simulink model "microduck_nonlinear_state_feedback"  (R2026b)
settings: Solver=ode15s  StopTime=r.test.duration  MaxStep=r.p.cfg.sim.maxStep  RelTol=r.p.cfg.sim.relTol  AbsTol=r.p.cfg.sim.absTol
PreLoadFcn:
  | root=fileparts(get_param(bdroot,'FileName')); addpath(root,fullfile(root,'helpers')); md_expanded_cache;
PostLoadFcn:
  | md_sf_apply(bdroot);
InitFcn:
  | md_sf_apply(bdroot);
model workspace (MAT data in the model file):
  G11 = [-0.6  0; 0  -0.6]
  G12 = -12
  G13 = -4000
  G14 = [-0.6  0; 0  -0.6]
  G15 = -12
  G16 = -4000
  G17 = [-0.6  0; 0  -0.6]
  G18 = -12
  G19 = -4000
  G20 = [-0.6  0; 0  -0.6]
  G21 = -12
  G22 = -4000
  G23 = [-0.6  0; 0  -0.6]
  G24 = -12
  G25 = -4000
  G26 = [-0.6  0; 0  -0.6]
  G27 = -12
  G28 = -4000
  G29 = [-0.6  0; 0  -0.6]
  G30 = -12
  G31 = -4000
  G32 = [-0.6  0; 0  -0.6]
  G33 = -12
  G34 = -4000
  G35 = [0  0  0  0  0  0  0  0; 0  0  0  0  0  0  0  0; 0  0  0  0  0  0  0  0; 0  0  0  0  0  0  0  0; 0  0  0  0  0  0  0  0; 0  0  0  0  0  0  0  0; 1  0  0  0  0  0  0  0; 0  1  0  0  0  0  0  0; 0  0  1  0  0  0  0  0; 0  0  0  1  0  0  0  0; 0  0  0  0  1  0  0  0; 0  0  0  0  0  1  0  0; 0  0  0  0  0  0  1  0; 0  0  0  0  0  0  0  1]
  G36 = [0  0  0  0  0  0  0  0; 0  0  0  0  0  0  0  0; 0  0  0  0  0  0  0  0; 0  0  0  0  0  0  0  0; 0  0  0  0  0  0  0  0; 0  0  0  0  0  0  0  0; 0.053  0  0  0  0  0  0  0; 0  0.053  0  0  0  0  0  0; 0  0  0.053  0  0  0  0  0; 0  0  0  0.053  0  0  0  0; 0  0  0  0  0.053  0  0  0; 0  0  0  0  0  0.053  0  0; 0  0  0  0  0  0  0.053  0; 0  0  0  0  0  0  0  0.053]
  G39 = [33.3333333333  0  0  0  0  0  0  0; 0  33.3333333333  0  0  0  0  0  0; 0  0  33.3333333333  0  0  0  0  0; 0  0  0  33.3333333333  0  0  0  0; 0  0  0  0  33.3333333333  0  0  0; 0  0  0  0  0  33.3333333333  0  0; 0  0  0  0  0  0  33.3333333333  0; 0  0  0  0  0  0  0  33.3333333333]
  G40 = [0  0  0  0  0  0  1  0  0  0  0  0  0  0; 0  0  0  0  0  0  0  1  0  0  0  0  0  0; 0  0  0  0  0  0  0  0  1  0  0  0  0  0; 0  0  0  0  0  0  0  0  0  1  0  0  0  0; 0  0  0  0  0  0  0  0  0  0  1  0  0  0; 0  0  0  0  0  0  0  0  0  0  0  1  0  0; 0  0  0  0  0  0  0  0  0  0  0  0  1  0; 0  0  0  0  0  0  0  0  0  0  0  0  0  1]
  G41 = [0  0  0  0  0  0  1  0  0  0  0  0  0  0; 0  0  0  0  0  0  0  1  0  0  0  0  0  0; 0  0  0  0  0  0  0  0  1  0  0  0  0  0; 0  0  0  0  0  0  0  0  0  1  0  0  0  0; 0  0  0  0  0  0  0  0  0  0  1  0  0  0; 0  0  0  0  0  0  0  0  0  0  0  1  0  0; 0  0  0  0  0  0  0  0  0  0  0  0  1  0; 0  0  0  0  0  0  0  0  0  0  0  0  0  1]
  Kd_servo = [0  0  0  0  0  0  0  0; 0  0  0  0  0  0  0  0; 0  0  0  0  0  0  0  0; 0  0  0  0  0  0  0  0; 0  0  0  0  0  0  0  0; 0  0  0  0  0  0  0  0; 0  0  0  0  0  0  0  0; 0  0  0  0  0  0  0  0]
  Kp_servo = [0.55  0  0  0  0  0  0  0; 0  0.55  0  0  0  0  0  0; 0  0  0.55  0  0  0  0  0; 0  0  0  0.55  0  0  0  0; 0  0  0  0  0.55  0  0  0; 0  0  0  0  0  0.55  0  0; 0  0  0  0  0  0  0.55  0; 0  0  0  0  0  0  0  0.55]
  c10 = 0
  c11 = 0
  c13 = 0
  c14 = 0
  c16 = 0
  c17 = 0
  c19 = 0
  c20 = 0
  c22 = 0
  c23 = 0
  c25 = 0
  c26 = 0
  c4 = 0
  c5 = 0
  c7 = 0
  c8 = 0
  g_world = [0; 0; -9.81]
  push_wrench = [1; 0; 0; 0; 0; 0]
  r.p.cfg.robot.gravity = [0; 0; -9.81]
  r.p.cfg.robot.hipHalfSpacing = 0.04
  r.p.cfg.robot.hipPitchDrop = 0.01
  r.p.cfg.robot.thighLength = 0.05
  r.p.cfg.robot.shinLength = 0.05
  r.p.cfg.robot.thighWidth = 0.025
  r.p.cfg.robot.shinWidth = 0.022
  r.p.cfg.robot.footLength = 0.054
  r.p.cfg.robot.footWidth = 0.041
  r.p.cfg.robot.footThickness = 0.012
  r.p.cfg.robot.soleDepth = 0.018
  r.p.cfg.robot.torsoDimensions = [0.09; 0.1; 0.14]
  r.p.cfg.robot.imuOffset = [0; 0; 0.05]
  r.p.cfg.robot.torsoCOM = [0; 0; 0.055]
  r.p.cfg.robot.carrierDimensions = [0.025; 0.025; 0.02]
  r.p.cfg.robot.massTorso = 0.5045154
  r.p.cfg.robot.massCarrier = 0.0287231
  r.p.cfg.robot.massThigh = 0.04315
  r.p.cfg.robot.massShin = 0.0215844
  r.p.cfg.robot.massFoot = 0.02646535
  r.p.cfg.robot.standingJointDeg = [0; -20; 40; -20; 0; -20; 40; -20]
  r.p.cfg.servo.kp = [0.55; 0.55; 0.55; 0.55; 0.55; 0.55; 0.55; 0.55]
  r.p.cfg.servo.kd = [0; 0; 0; 0; 0; 0; 0; 0]
  r.p.cfg.servo.timeConstant = [0.03; 0.03; 0.03; 0.03; 0.03; 0.03; 0.03; 0.03]
  r.p.cfg.servo.maxTorque = [0.6; 0.6; 0.6; 0.6; 0.6; 0.6; 0.6; 0.6]
  r.p.cfg.servo.jointDamping = [0.053; 0.053; 0.053; 0.053; 0.053; 0.053; 0.053; 0.053]
  r.p.cfg.servo.minCommandDeg = [-20.0535228296; -57.2957795131; 2.86478897565; -45.8366236105; -20.0535228296; -57.2957795131; 2.86478897565; -45.8366236105]
  r.p.cfg.servo.maxCommandDeg = [20.0535228296; 34.3774677078; 85.9436692696; 45.8366236105; 20.0535228296; 34.3774677078; 85.9436692696; 45.8366236105]
  r.p.cfg.contact.stiffness = 4000
  r.p.cfg.contact.damping = 12
  r.p.cfg.contact.friction = 0.6
  r.p.cfg.contact.frictionVelocity = 0.005
  r.p.cfg.sim.sampleTime = 0.02
  r.p.cfg.sim.stopTime = 3
  r.p.cfg.sim.maxStep = 0.002
  r.p.cfg.sim.relTol = 1e-06
  r.p.cfg.sim.absTol = 1e-08
  r.p.cfg.stop.enabled = 1
  r.p.cfg.stop.maxTiltDeg = 20
  r.p.cfg.stop.minHipHeight = 0.06
  r.p.cfg.measurements.includeJointVelocity = 0
  r.p.g = [0; 0; -9.81]
  r.p.nq = 14
  r.p.S = [0  0  0  0  0  0  0  0; 0  0  0  0  0  0  0  0; 0  0  0  0  0  0  0  0; 0  0  0  0  0  0  0  0; 0  0  0  0  0  0  0  0; 0  0  0  0  0  0  0  0; 1  0  0  0  0  0  0  0; 0  1  0  0  0  0  0  0; 0  0  1  0  0  0  0  0; 0  0  0  1  0  0  0  0; 0  0  0  0  1  0  0  0; 0  0  0  0  0  1  0  0; 0  0  0  0  0  0  1  0; 0  0  0  0  0  0  0  1]
  r.p.kp = [0.55; 0.55; 0.55; 0.55; 0.55; 0.55; 0.55; 0.55]
  r.p.kd = [0; 0; 0; 0; 0; 0; 0; 0]
  r.p.Ta = [0.03; 0.03; 0.03; 0.03; 0.03; 0.03; 0.03; 0.03]
  r.p.tauMax = [0.6; 0.6; 0.6; 0.6; 0.6; 0.6; 0.6; 0.6]
  r.p.bjoint = [0.053; 0.053; 0.053; 0.053; 0.053; 0.053; 0.053; 0.053]
  r.p.jointMin = [-0.35; -1; 0.05; -0.8; -0.35; -1; 0.05; -0.8]
  r.p.jointMax = [0.35; 0.6; 1.5; 0.8; 0.35; 0.6; 1.5; 0.8]
  r.p.kn = 4000
  r.p.cn = 12
  r.p.mu = 0.6
  r.p.vs = 0.005
  r.p.imuOffset = [0; 0; 0.05]
  r.p.parent = [0 1 2 3 4 1 6 7 8]
  r.p.jointIndex = [0 7 8 9 10 11 12 13 14]
  r.p.axis = [0  1  0  0  0  1  0  0  0; 0  0  1  1  1  0  1  1  1; 0  0  0  0  0  0  0  0  0]
  r.p.offset = [0  0  0  0  0  0  0  0  0; 0  0.04  0  0  0  -0.04  0  0  0; 0  0  -0.01  -0.05  -0.05  0  -0.01  -0.05  -0.05]
  r.p.mass = [0.5045154 0.0287231 0.04315 0.0215844 0.02646535 0.0287231 0.04315 0.0215844 0.02646535]
  r.p.com = [0  0  0  0  0  0  0  0  0; 0  0  0  0  0  0  0  0  0; 0.055  -0.005  -0.025  -0.025  -0.012  -0.005  -0.025  -0.025  -0.012]
  r.p.inertia = reshape([0.00124447132 0 0 0 0.001164589715 0 0 0 0.000760977395 2.45343145833e-06 0 0 0 2.45343145833e-06 0 0 0 2.99198958333e-06 1.12369791667e-05 0 0 0 1.12369791667e-05 0 0 0 4.49479166667e-06 5.3673208e-06 0 0 0 5.3673208e-06 0 0 0 1.7411416e-06 4.02493864583e-06 0 0 0 6.74866425e-06 0 0 0 1.01384344958e-05 2.45343145833e-06 0 0 0 2.45343145833e-06 0 0 0 2.99198958333e-06 1.12369791667e-05 0 0 0 1.12369791667e-05 0 0 0 4.49479166667e-06 5.3673208e-06 0 0 0 5.3673208e-06 0 0 0 1.7411416e-06 4.02493864583e-06 0 0 0 6.74866425e-06 0 0 0 1.01384344958e-05], [3 3 9])
  r.p.footBodies = [5 9]
  r.p.corners = [-0.027  -0.027  0.027  0.027; -0.0205  0.0205  -0.0205  0.0205; -0.018  -0.018  -0.018  -0.018]
  r.p.qnom = [0; 0; 0.121741068879; 0; 0; 0; 0; -0.349065850399; 0.698131700798; -0.349065850399; 0; -0.349065850399; 0.698131700798; -0.349065850399]
  r.p.trimResidual = 3.34843264227e-13
  r.p.trimNormal = [0.86015562883; 0.86015562883; 0.96538996892; 0.96538996892; 0.86015562883; 0.86015562883; 0.96538996892; 0.96538996892]
  r.p.xeq = [0; 0; 0.121741054404; 0; 0.00048719603821; 6.28632250353e-17; 0; -0.349065850399; 0.698131700798; -0.349065850399; 0; -0.349065850399; 0.698131700798; -0.349065850399; 0; 0; 0; 0; 0; 0; 0; 0; 0; 0; 0; 0; 0; 0; 5.52116353176e-16; 7.90529085794e-05; -0.0506100270862; 0.00565215320243; 5.52116353176e-16; 7.90529085794e-05; -0.0506100270862; 0.00565215320243]
  r.p.ueq = [1.00384791487e-15; -0.348922117838; 0.606113469732; -0.338789208213; 1.00384791487e-15; -0.348922117838; 0.606113469732; -0.338789208213]
  r.lin.A = [0 0 0 0 0 0 0 0 0 0 0 0 ... (1296 elements, 36x36)]
  r.lin.B = [0  0  0  0  0  0  0  0; 0  0  0  0  0  0  0  0; 0  0  0  0  0  0  0  0; 0  0  0  0  0  0  0  0; 0  0  0  0  0  0  0  0; 0  0  0  0  0  0  0  0; 0  0  0  0  0  0  0  0; 0  0  0  0  0  0  0  0; 0  0  0  0  0  0  0  0; 0  0  0  0  0  0  0  0; 0  0  0  0  0  0  0  0; 0  0  0  0  0  0  0  0; 0  0  0  0  0  0  0  0; 0  0  0  0  0  0  0  0; 0  0  0  0  0  0  0  0; 0  0  0  0  0  0  0  0; 0  0  0  0  0  0  0  0; 0  0  0  0  0  0  0  0; 0  0  0  0  0  0  0  0; 0  0  0  0  0  0  0  0; 0  0  0  0  0  0  0  0; 0  0  0  0  0  0  0  0; 0  0  0  0  0  0  0  0; 0  0  0  0  0  0  0  0; 0  0  0  0  0  0  0  0; 0  0  0  0  0  0  0  0; 0  0  0  0  0  0  0  0; 0  0  0  0  0  0  0  0; 18.3333333333  0  0  0  0  0  0  0; 0  18.3333333328  0  0  0  0  0  0; 0  0  18.3333333339  0  0  0  0  0; 0  0  0  18.3333333328  0  0  0  0; 0  0  0  0  18.3333333333  0  0  0; 0  0  0  0  0  18.3333333328  0  0; 0  0  0  0  0  0  18.3333333339  0; 0  0  0  0  0  0  0  18.3333333328]
  r.lin.C = [0  0  0  0  0  0  0  0  0  0  0  0  0  0  0  0  0  -0.000487196018936  0  1  0  0  0  0  0  0  0  0  0  0  0  0  0  0  0  0; 0  0  0  0  0  0  0  0  0  0  0  0  0  0  0  0  0  6.28632175747e-17  1  5.73971850987e-36  0  0  0  0  0  0  0  0  0  0  0  0  0  0  0  0; 0  0  0  0  0  0  0  0  0  0  0  0  0  0  0  0  0  0.99999988132  -6.28632250353e-17  0  0  0  0  0  0  0  0  0  0  0  0  0  0  0  0  0; 0  0  9265.46457746  0  130.165054704  -6.84001466578e-08  -2.07256087292e-09  69.3951978499  144.565706863  64.1932730965  -2.10595429984e-09  69.3951978499  144.565706863  64.1932730965  74.0137947271  0  27.7963937321  6.20163642662e-11  -8.63881750136  -1.78676518026e-10  2.86229373536e-10  -5.26342586956  -0.830679547445  0.178354369236  2.57172755314e-10  -5.26342586956  -0.830679547439  0.178354369236  0  24.7927989485  -21.5530077617  -12.2808996456  0  24.7927989485  -21.5530077617  -12.2808996456; 0  0  -7.82627372827e-11  -1.15367357622e-10  1.01085418767e-08  272.89136386  112.119374165  10.1316970194  18.6847145316  9.9177480342  112.119374165  -10.1316970296  -18.6847145316  -9.9177480442  8.21255251386e-14  515.113047543  -3.2086916701e-11  0.947725865768  -3.57478340115e-11  63.6596220389  32.5958842775  -0.557372026813  -0.482069576678  0.0855967928727  32.5958842776  0.55737202677  0.482069576771  -0.0855967928114  -15.5718784225  -0.992982191643  3.13034753722  -2.99186872359  -15.5718784225  0.992982191643  -3.13034753722  2.99186872359; 0  0  -13045.3812466  0  -291.511055468  1.00364161426e-07  4.4408920985e-09  -145.399577004  -260.915887701  -143.957256833  4.4408920985e-09  -145.399577003  -260.915887701  -143.957256832  -165.916252803  0  -39.1361437391  8.881784197e-10  19.3664195969  0  8.881784197e-10  7.18267224187  7.99488262881  -1.40613470379  0  7.18267224276  7.99488262881  -1.40613470467  0  31.5292775177  -63.6564564429  46.5139879342  0  31.5292775177  -63.6564564429  46.5139879342]
  r.lin.D = [0  0  0  0  0  0  0  0; 0  0  0  0  0  0  0  0; 0  0  0  0  0  0  0  0; 0  0  0  0  0  0  0  0; 0  0  0  0  0  0  0  0; 0  0  0  0  0  0  0  0]
  r.lin.C_with_joint_angles = [0 0 0 0 0 0 0 0 0 0 0 0 ... (504 elements, 14x36)]
  r.lin.D_with_joint_angles = [0  0  0  0  0  0  0  0; 0  0  0  0  0  0  0  0; 0  0  0  0  0  0  0  0; 0  0  0  0  0  0  0  0; 0  0  0  0  0  0  0  0; 0  0  0  0  0  0  0  0; 0  0  0  0  0  0  0  0; 0  0  0  0  0  0  0  0; 0  0  0  0  0  0  0  0; 0  0  0  0  0  0  0  0; 0  0  0  0  0  0  0  0; 0  0  0  0  0  0  0  0; 0  0  0  0  0  0  0  0; 0  0  0  0  0  0  0  0]
  r.lin.C_measurements = [0 0 0 0 0 0 0 0 0 0 0 0 ... (504 elements, 14x36)]
  r.lin.D_measurements = [0  0  0  0  0  0  0  0; 0  0  0  0  0  0  0  0; 0  0  0  0  0  0  0  0; 0  0  0  0  0  0  0  0; 0  0  0  0  0  0  0  0; 0  0  0  0  0  0  0  0; 0  0  0  0  0  0  0  0; 0  0  0  0  0  0  0  0; 0  0  0  0  0  0  0  0; 0  0  0  0  0  0  0  0; 0  0  0  0  0  0  0  0; 0  0  0  0  0  0  0  0; 0  0  0  0  0  0  0  0; 0  0  0  0  0  0  0  0]
  r.lin.xeq = [0; 0; 0.121741054404; 0; 0.00048719603821; 6.28632250353e-17; 0; -0.349065850399; 0.698131700798; -0.349065850399; 0; -0.349065850399; 0.698131700798; -0.349065850399; 0; 0; 0; 0; 0; 0; 0; 0; 0; 0; 0; 0; 0; 0; 5.52116353176e-16; 7.90529085794e-05; -0.0506100270862; 0.00565215320243; 5.52116353176e-16; 7.90529085794e-05; -0.0506100270862; 0.00565215320243]
  r.lin.ueq = [1.00384791487e-15; -0.348922117838; 0.606113469732; -0.338789208213; 1.00384791487e-15; -0.348922117838; 0.606113469732; -0.338789208213]
  r.lin.yeq = [0; 0; 0; -0.00477939294573; 2.9613909167e-15; 9.80999883575]
  r.lin.yeq_measurements = [0; 0; 0; -0.00477939294573; 2.9613909167e-15; 9.80999883575; 0; -0.349065850399; 0.698131700798; -0.349065850399; 0; -0.349065850399; 0.698131700798; -0.349065850399]
  r.lin.stateScale = [0.01; 0.01; 0.01; 0.1; 0.1; 0.1; 0.1; 0.1; 0.1; 0.1; 0.1; 0.1; 0.1; 0.1; 0.1; 0.1; 0.1; 1; 1; 1; 1; 1; 1; 1; 1; 1; 1; 1; 0.1; 0.1; 0.1; 0.1; 0.1; 0.1; 0.1; 0.1]
  r.lin.controlSampleTime = 0.02
  r.aux.E = [0  0  0  0  0  0; 0  0  0  0  0  0; 0  0  0  0  0  0; 0  0  0  0  0  0; 0  0  0  0  0  0; 0  0  0  0  0  0; 0  0  0  0  0  0; 0  0  0  0  0  0; 0  0  0  0  0  0; 0  0  0  0  0  0; 0  0  0  0  0  0; 0  0  0  0  0  0; 0  0  0  0  0  0; 0  0  0  0  0  0; 2.99982286451  -1.39842679811e-16  0.177414688657  -4.57651764544e-15  -30.0277204497  6.50739104523e-15; -1.58268629198e-16  2.89225820935  6.70083365122e-17  26.4522242149  3.51536253633e-15  -2.99721816856; 0.177414688663  8.37728579002e-17  1.49617665797  1.51751719319e-15  -1.96848927847  1.08542064426e-15; 6.08932332349e-15  -2.9843307487  6.98022045066e-16  -46.5047890403  -1.8610446411e-13  1033.95442638; -30.0277204497  3.01733642702e-15  -1.9684892784  9.66057478592e-14  670.762570803  -1.79597476519e-13; -2.99085236462e-15  26.4522273543  1.22764163289e-15  571.194337556  6.97130001697e-14  -46.7830781998; 4.28916538281e-15  -58.9426085695  -3.230112201e-15  -867.400266402  -9.48911648967e-14  29.6379320526; 93.8758569341  20.513888201  31.4835453095  429.750563248  -1381.35416373  -794.127195927; -48.639015031  -44.7564909477  -63.6327672593  -957.446876757  541.099997319  595.256445506; -27.6741686092  33.1017153167  46.5274762001  722.046276778  308.318673607  358.193155987; 4.44518421763e-15  -58.9426085695  -2.95924669915e-15  -867.400266402  -9.69858375627e-14  29.6379320526; 93.8758569341  -20.513888201  31.4835453095  -429.750563248  -1381.35416373  794.127195927; -48.639015031  44.7564909477  -63.6327672593  957.446876757  541.099997319  -595.256445506; -27.6741686092  -33.1017153167  46.5274762001  -722.046276778  308.318673607  -358.193155987; 0  0  0  0  0  0; 0  0  0  0  0  0; 0  0  0  0  0  0; 0  0  0  0  0  0; 0  0  0  0  0  0; 0  0  0  0  0  0; 0  0  0  0  0  0; 0  0  0  0  0  0]
  r.aux.Fw = [0  0  0  0  0  0; 0  0  0  0  0  0; 0  0  0  0  0  0; 1.49835005027  0  0.0782612723698  0  3.51137069423  0; 2.66705636347e-18  1.56957414393  9.97031711871e-17  -2.1086255103  -9.94861602458e-17  -0.632877334553; 0.178876169343  0  1.49626291615  0  -1.98311843072  0; 0  0  0  0  0  0; 0  0  0  0  0  0; 0  0  0  0  0  0; 0  0  0  0  0  0; 0  0  0  0  0  0; 0  0  0  0  0  0; 0  0  0  0  0  0; 0  0  0  0  0  0]
  r.feedback.K = [8.70410247674e-16 -0.000482616394029 -0.000818546928294 -0.00100799621853 -3.20893583014e-15 -0.000482616394022 -0.000818546928299 -0.00100799621853 3.94214592664e-14 -0.0216180096191 -0.0366654667942 -0.0451515369514 ... (264 elements, 8x33)]
  r.feedback.poles = [-0.173706973501+0.0790896944051i; -0.173706973501-0.0790896944051i; -0.014115987547+0.0894236107172i; -0.014115987547-0.0894236107172i; 0.672250176228+0.561912229918i; 0.672250176228-0.561912229918i; -0.0822703613827+0.0594677475137i; -0.0822703613827-0.0594677475137i; 0.0992828819218+0i; 0.891684694096+0i; 0.886920436717+0i; 0.735487634412+0.114439990771i; 0.735487634412-0.114439990771i; 0.717373000186+0.112026826557i; 0.717373000186-0.112026826557i; 0.976285709758+0i; 0.980198673307+0i; 0.721801481118+0.118511971968i; 0.721801481118-0.118511971968i; 0.482156928981+0i; 0.480371127775+0i; 0.492850316995+0i; 0.515715029329+0i; 0.514305187301+0i; 2.94698823164e-09+0i; -5.41379190099e-16+0i; 1.47117542566e-16+0i; 1.11020150478e-17+9.9609496806e-17i; 1.11020150478e-17-9.9609496806e-17i; -2.28360718307e-17+3.66102795761e-17i; -2.28360718307e-17-3.66102795761e-17i; 2.99664398283e-17+2.17653008708e-17i; 2.99664398283e-17-2.17653008708e-17i]
  r.feedback.requestedPoles = [-0.173706973501+0.0790896944051i; -0.173706973501-0.0790896944051i; -0.014115987547+0.0894236107172i; -0.014115987547-0.0894236107172i; 0.672250176228+0.561912229918i; 0.672250176228-0.561912229918i; -0.0822703613827+0.0594677475137i; -0.0822703613827-0.0594677475137i; 0.0992828819218+0i; 0.891684694096+0i; 0.735487634412+0.114439990771i; 0.735487634412-0.114439990771i; 0.717373000186+0.112026826557i; 0.717373000186-0.112026826557i; 0.721801481118+0.118511971968i; 0.721801481118-0.118511971968i; 0.482156928981+0i; 0.480371127775+0i; 0.492850316995+0i; 0.515715029329+0i; 0.514305187301+0i; 2.9469884e-09+0i; 5.84077967475e-15+0i; -2.65521112042e-15+2.05477564382e-15i; -2.65521112042e-15-2.05477564382e-15i; 3.09349036794e-15+0i; 9.13638941562e-16+0i; -4.87155219894e-16+0i; 1.66967134563e-16+2.25567004766e-16i; 1.66967134563e-16-2.25567004766e-16i; 0.886920436717+0i; 0.976285709758+0i; 0.980198673307+0i]
  r.feedback.assignedSlowPoles = [0.886920436717; 0.976285709758; 0.980198673307]
  r.feedback.retainedFastPoleCount = 30
  r.feedback.poleMatchError = 1.58095758707e-13
  r.feedback.placementPrecision = 15
  r.feedback.radius = 0.980198673307
  r.feedback.reference = [0; 0]
  r.feedback.maxCorrectionRad = 0.13962634016
  r.feedback.sampleTime = 0.02
  r.observer.Ad = [-0.226035158295 0.0607901151539 1.20046417563e-11 -1.4732593899e-11 -0.156351729745 0.138229107162 0.0857639497085 -1.47317675914e-11 -0.156351729733 0.138229107138 0.0857639497232 1.19581922834 ... (1089 elements, 33x33)]
  r.observer.Bd = [-1.57872286761e-12 -2.75043555489e-12 -0.0544924598499 0.0922096305921 -0.0255771207666 0.0488604655049 -0.0163542439887 0.087766164084 0.0255771207875 -0.0488604655276 0.016354243994 1.82708257098e-11 ... (264 elements, 33x8)]
  r.observer.C = [0 0 0 9.44491801984 -7.97785293402e-14 -13.2980440841 0 0 0 0 0 0 ... (462 elements, 14x33)]
  r.observer.D = [0  0  0  0  0  0  0  0; 0  0  0  0  0  0  0  0; 0  0  0  0  0  0  0  0; 0  0  0  0  0  0  0  0; 0  0  0  0  0  0  0  0; 0  0  0  0  0  0  0  0; 0  0  0  0  0  0  0  0; 0  0  0  0  0  0  0  0; 0  0  0  0  0  0  0  0; 0  0  0  0  0  0  0  0; 0  0  0  0  0  0  0  0; 0  0  0  0  0  0  0  0; 0  0  0  0  0  0  0  0; 0  0  0  0  0  0  0  0]
  r.observer.L = [-7.01418682646e-12 8.04628712517e-11 0.0643927661333 0.24278751739 0.0372639622641 -0.0756135571544 0.0275453071133 0.242787517394 -0.0372639605356 0.07561355728 -0.0275453090267 5.98286207219e-10 ... (462 elements, 33x14)]
  r.observer.errorMatrix = [-0.251020245761 0.799832731146 2.38563787379e-09 7.04126391556e-09 2.62313977309 0.267993545053 -3.41200716347 7.0849640839e-09 2.62313976989 0.267993551207 -3.41200716574 3.40012488569 ... (1089 elements, 33x33)]
  r.observer.poles = [-0.173706973501+0.0790896944051i; -0.173706973501-0.0790896944051i; -0.014115987547+0.0894236107172i; -0.014115987547-0.0894236107172i; -0.0822703613827+0.0594677475137i; -0.0822703613827-0.0594677475137i; 0.0992828819218+0i; 0.717373000186+0.112026826557i; 0.717373000186-0.112026826557i; 0.721801481118+0.118511971968i; 0.721801481118-0.118511971968i; 0.670320046036+0i; 0.482156928981+0i; 0.582748252374+0i; 0.59452054797+0i; 0.631283645507+0i; 0.657046819815+0i; 0.644036421083+0i; 0.618783391806+0i; 0.606530659713+0i; 0.480371127775+0i; 0.492850316995+0i; 0.514305187301+0i; 0.515715029329+0i; 2.94698765516e-09+0i; 1.91663560711e-14+0i; -6.86720396472e-15+0i; -3.48279432533e-16+9.37889198838e-16i; -3.48279432533e-16-9.37889198838e-16i; 7.85859192971e-16+3.70757158126e-16i; 7.85859192971e-16-3.70757158126e-16i; -2.4574281643e-16+0i; 2.80192628595e-16+0i]
  r.observer.continuousA = [0 0 0 0 0 0 0 0 0 0 0 2088.98331426 ... (1089 elements, 33x33)]
  r.observer.continuousB = [0  0  0  0  0  0  0  0; 0  0  0  0  0  0  0  0; 0  0  0  0  0  0  0  0; 0  0  0  0  0  0  0  0; 0  0  0  0  0  0  0  0; 0  0  0  0  0  0  0  0; 0  0  0  0  0  0  0  0; 0  0  0  0  0  0  0  0; 0  0  0  0  0  0  0  0; 0  0  0  0  0  0  0  0; 0  0  0  0  0  0  0  0; 0  0  0  0  0  0  0  0; 0  0  0  0  0  0  0  0; 0  0  0  0  0  0  0  0; 0  0  0  0  0  0  0  0; 0  0  0  0  0  0  0  0; 0  0  0  0  0  0  0  0; 0  0  0  0  0  0  0  0; 0  0  0  0  0  0  0  0; 0  0  0  0  0  0  0  0; 0  0  0  0  0  0  0  0; 0  0  0  0  0  0  0  0; 0  0  0  0  0  0  0  0; 0  0  0  0  0  0  0  0; 0  0  0  0  0  0  0  0; 183.333333333  0  0  0  0  0  0  0; 0  183.333333328  0  0  0  0  0  0; 0  0  183.333333339  0  0  0  0  0; 0  0  0  183.333333328  0  0  0  0; 0  0  0  0  183.333333333  0  0  0; 0  0  0  0  0  183.333333328  0  0; 0  0  0  0  0  0  183.333333339  0; 0  0  0  0  0  0  0  183.333333328]
  r.observer.y0 = [0; 0; 0; -0.00477939294573; 2.9613909167e-15; 9.80999883575; 0; -0.349065850399; 0.698131700798; -0.349065850399; 0; -0.349065850399; 0.698131700798; -0.349065850399]
  r.observer.yScale = [1; 1; 1; 9.81; 9.81; 9.81; 0.1; 0.1; 0.1; 0.1; 0.1; 0.1; 0.1; 0.1]
  r.observer.keep = [3 5 6 7 8 9 10 11 12 13 14 15 16 17 18 19 20 21 22 23 24 25 26 27 28 29 30 31 32 33 34 35 36]
  r.observer.S = [0.01 0 0 0 0 0 0 0 0 0 0 0 ... (1089 elements, 33x33)]
  r.observer.settings.initialAngleErrorDeg = [0.5; 1]
  r.observer.settings.slowModeCutoffRate = 15
  r.observer.settings.firstDecayRate = 20
  r.observer.settings.decayRateSpacing = 1
  r.observer.settings.initialEstimateDelta = [0; 0; 0; 0; 0.0174532925199; 0.00872664625997; 0; 0; 0; 0; 0; 0; 0; 0; 0; 0; 0; 0; 0; 0; 0; 0; 0; 0; 0; 0; 0; 0; 0; 0; 0; 0; 0; 0; 0; 0]
  r.observer.sampleTime = 0.02
  r.observer.requestedSlowPoles = [0.670320046036 0.657046819815 0.644036421083 0.631283645507 0.618783391806 0.606530659713 0.59452054797 0.582748252374]
  r.observer.retainedFastPoleCount = 25
  r.observer.placementPrecision = 14
  r.test.duration = 3
  r.test.pushForce = [1; 0; 0]
  r.test.pushMoment = [0; 0; 0]
  r.test.pushCentre = 0.2
  r.test.pushWidth = 0.02
  r.test.pushEnabled = 1
  r.test.pushPointBody = [0; 0; 0]
  r.H = [0  0  1  0  0  0  0  0  0  0  0  0  0  0  0  0  0  0  0  0  0  0  0  0  0  0  0  0  0  0  0  0  0; 0  1  0  0  0  0  0  0  0  0  0  0  0  0  0  0  0  0  0  0  0  0  0  0  0  0  0  0  0  0  0  0  0]
  r.sharedConfiguration.test.duration = 3
  r.sharedConfiguration.test.pushForce = [1; 0; 0]
  r.sharedConfiguration.test.pushMoment = [0; 0; 0]
  r.sharedConfiguration.test.pushCentre = 0.2
  r.sharedConfiguration.test.pushWidth = 0.02
  r.sharedConfiguration.sampleTime = 0.02
  r.sharedConfiguration.observer.initialAngleErrorDeg = [0.5; 1]
  r.sharedConfiguration.observer.slowModeCutoffRate = 15
  r.sharedConfiguration.observer.firstDecayRate = 20
  r.sharedConfiguration.observer.decayRateSpacing = 1
  r.sharedConfiguration.robot.gravity = [0; 0; -9.81]
  r.sharedConfiguration.robot.hipHalfSpacing = 0.04
  r.sharedConfiguration.robot.hipPitchDrop = 0.01
  r.sharedConfiguration.robot.thighLength = 0.05
  r.sharedConfiguration.robot.shinLength = 0.05
  r.sharedConfiguration.robot.thighWidth = 0.025
  r.sharedConfiguration.robot.shinWidth = 0.022
  r.sharedConfiguration.robot.footLength = 0.054
  r.sharedConfiguration.robot.footWidth = 0.041
  r.sharedConfiguration.robot.footThickness = 0.012
  r.sharedConfiguration.robot.soleDepth = 0.018
  r.sharedConfiguration.robot.torsoDimensions = [0.09; 0.1; 0.14]
  r.sharedConfiguration.robot.imuOffset = [0; 0; 0.05]
  r.sharedConfiguration.robot.torsoCOM = [0; 0; 0.055]
  r.sharedConfiguration.robot.carrierDimensions = [0.025; 0.025; 0.02]
  r.sharedConfiguration.robot.massTorso = 0.5045154
  r.sharedConfiguration.robot.massCarrier = 0.0287231
  r.sharedConfiguration.robot.massThigh = 0.04315
  r.sharedConfiguration.robot.massShin = 0.0215844
  r.sharedConfiguration.robot.massFoot = 0.02646535
  r.sharedConfiguration.robot.standingJointDeg = [0; -20; 40; -20; 0; -20; 40; -20]
  r.sharedConfiguration.servo.kp = [0.55; 0.55; 0.55; 0.55; 0.55; 0.55; 0.55; 0.55]
  r.sharedConfiguration.servo.kd = [0; 0; 0; 0; 0; 0; 0; 0]
  r.sharedConfiguration.servo.timeConstant = [0.03; 0.03; 0.03; 0.03; 0.03; 0.03; 0.03; 0.03]
  r.sharedConfiguration.servo.maxTorque = [0.6; 0.6; 0.6; 0.6; 0.6; 0.6; 0.6; 0.6]
  r.sharedConfiguration.servo.jointDamping = [0.053; 0.053; 0.053; 0.053; 0.053; 0.053; 0.053; 0.053]
  r.sharedConfiguration.servo.minCommandDeg = [-20.0535228296; -57.2957795131; 2.86478897565; -45.8366236105; -20.0535228296; -57.2957795131; 2.86478897565; -45.8366236105]
  r.sharedConfiguration.servo.maxCommandDeg = [20.0535228296; 34.3774677078; 85.9436692696; 45.8366236105; 20.0535228296; 34.3774677078; 85.9436692696; 45.8366236105]
  r.sharedConfiguration.contact.stiffness = 4000
  r.sharedConfiguration.contact.damping = 12
  r.sharedConfiguration.contact.friction = 0.6
  r.sharedConfiguration.contact.frictionVelocity = 0.005
  r.sharedConfiguration.feedback.assignedDecayRates = [6; 1; 1.2]
  r.sharedConfiguration.feedback.slowModeCutoffRate = 2.5
  r.sharedConfiguration.feedback.poleMatchTolerance = 1e-06
  r.sharedConfiguration.feedback.maxCorrectionDeg = 8
  r.sharedConfiguration.solver.maxStep = 0.002
  r.sharedConfiguration.solver.relTol = 1e-06
  r.sharedConfiguration.solver.absTol = 1e-08
  r.sharedConfiguration.validity.maxTiltDeg = 20
  r.sharedConfiguration.validity.minHipHeight = 0.06
  r.sharedVersion = 1
  r.mode = 'nonlinear'
  v_s2 = 2.5e-05
(part 1 of 5)
settings Model: Creator=parve  LastModifiedBy=parve

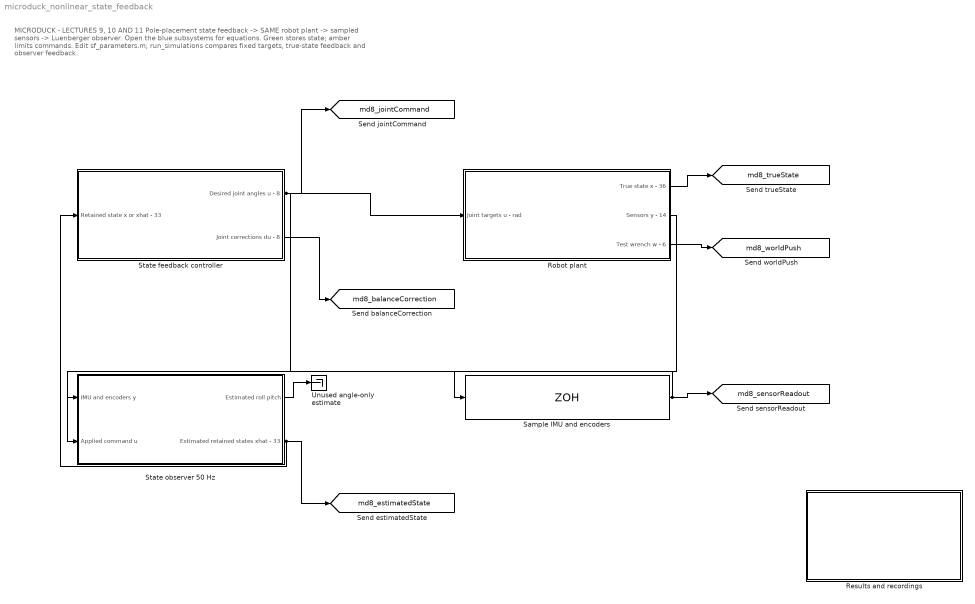
== system microduck_nonlinear_state_feedback ==
  note: MICRODUCK - LECTURES 9, 10 AND 11
      | Pole-placement state feedback -> SAME robot plant -> sampled sensors -> Luenberger observer.
      | Open the blue subsystems for equations. Green stores state; amber limits commands.
      | Edit sf_parameters.m; run_simulations compares fixed targets, true-state feedback and observer feedback.
  Results and recordings : Subsystem  Description=|
      | RESULTS AND RECORDINGS
      | 
      | Purpose: record signals for plotting and comparison. These blocks do not control the robot.
      | trueState: actual motion; estimatedState: observer output; jointCommand: applied targets.
      | sensorReadout, worldPush and balanceCorrection complete the experiment records.
      mask help:
      | RESULTS AND RECORDINGS
      |
      | Purpose: record signals for plotting and comparison. These blocks do not control the robot.
      | trueState: actual motion; estimatedState: observer output; jointCommand: applied targets.
      | sensorReadout, worldPush and balanceCorrection complete the experiment records.
      settings: OpenFcn=open_system(gcb,'force');
      mask Display: disp('Results and recordings');
  Robot plant : Subsystem  Description=|
      | ROBOT PLANT
      | 
      | Purpose: predict how the robot moves when its eight servo targets change.
      | Read the folders for motor torque, body motion, ground forces and sensors.
      | Inputs are desired joint angles; outputs are true states, sensor readings and the test push.
      mask help:
      | ROBOT PLANT
      |
      | Purpose: predict how the robot moves when its eight servo targets change.
      | Read the folders for motor torque, body motion, ground forces and sensors.
      | Inputs are desired joint angles; outputs are true states, sensor readings and the test push.
      settings: OpenFcn=open_system(gcb,'force');
      mask Display: disp('Robot plant');
  Sample IMU and encoders : ZeroOrderHold  Description=|  SampleTime=r.observer.sampleTime
      | Sample IMU and encoders
      | 
      | WHAT THIS BLOCK DOES
      | Samples the sensor signal every 0.02 s and holds that measurement between samples, representing the 50 Hz readout clock.
      | 
      | FOLDER CONTEXT
      | MICRODUCK BALANCE - START HERE
      | 
      | Follow the loop: state-feedback controller -> robot plant -> sampled sensors -> observer -> PID.
      | Open a folder for its purpose, signal meanings and equations. Green blocks store state; amber blocks limit signals.
      | The controller and observer update at 50 Hz. Results are recorded separately on the right.
  State feedback controller : Subsystem  Description=Lecture 9 pole-placement feedback. Normalize standing state deviations, apply -K, limit offsets, and add standing joint targets.
      settings: OpenFcn=open_system(gcb,'force');
      mask Display: disp('State feedback controller\nLecture 9: pole placement')
  State observer 50 Hz : Subsystem  Description=|
      | Lecture 10 Luenberger observer, sampled as in Lecture 11.
      | zhat[k+1]=Ad zhat[k]+Bd du[k]+L(yn[k]-Cn zhat[k]).
      | The same applied joint target is sent to both plant and observer.
      settings: OpenFcn=open_system(gcb,'force');
      mask Display: disp('State observer\nLuenberger pole placement')
  Unused angle-only estimate : Terminator
  tag scope: md8_balanceCorrection=global, md8_estimatedState=global, md8_jointCommand=global, md8_sensorReadout=global, md8_trueState=global, md8_worldPush=global
  wires:
  State feedback controller/1(Desired joint angles u - 8) -> Robot plant/1(Joint targets u - rad), State observer 50 Hz/2(Applied command u), [md8_jointCommand]
  State feedback controller/2(Joint corrections du - 8) -> [md8_balanceCorrection]
  Robot plant/1(True state x - 36) -> [md8_trueState]
  Robot plant/2(Sensors y - 14) -> Sample IMU and encoders/1
  Robot plant/3(Test wrench w - 6) -> [md8_worldPush]
  Sample IMU and encoders/1 -> State observer 50 Hz/1(IMU and encoders y), [md8_sensorReadout]
  State observer 50 Hz/2(Estimated retained states xhat - 33) -> State feedback controller/1(Retained state x or xhat - 33), [md8_estimatedState]
  State observer 50 Hz/1(Estimated roll pitch) -> Unused angle-only estimate/1

== system microduck_nonlinear_state_feedback/Results and recordings ==
  note: RESULTS AND RECORDINGS
      |
      | Purpose: record signals for plotting and comparison. These blocks do not control the robot.
      | trueState: actual motion; estimatedState: observer output; jointCommand: applied targets.
      | sensorReadout, worldPush and balanceCorrection complete the experiment records.
  balanceCorrection : ToWorkspace  VariableName=balanceCorrection  SaveFormat=Timeseries  SampleTime=-1
      settings: Description=|
      | balanceCorrection
      | 
      | WHAT THIS BLOCK DOES
      | Records the input as a MATLAB timeseries for plots and validation. It does not feed a control action back to the robot.
      | 
      | FOLDER CONTEXT
      | RESULTS AND RECORDINGS
      | 
      | Purpose: record signals for plotting and comparison. These blocks do not control the robot.
      | trueState: actual motion; estimatedState: observer output; jointCommand: applied targets.
      | sensorReadout, worldPush and balanceCorrection complete the experiment records.
  estimatedState : ToWorkspace  VariableName=estimatedState  SaveFormat=Timeseries  SampleTime=-1
      settings: Description=|
      | estimatedState
      | 
      | WHAT THIS BLOCK DOES
      | Records the input as a MATLAB timeseries for plots and validation. It does not feed a control action back to the robot.
      | 
      | FOLDER CONTEXT
      | RESULTS AND RECORDINGS
      | 
      | Purpose: record signals for plotting and comparison. These blocks do not control the robot.
      | trueState: actual motion; estimatedState: observer output; jointCommand: applied targets.
      | sensorReadout, worldPush and balanceCorrection complete the experiment records.
  jointCommand : ToWorkspace  VariableName=jointCommand  SaveFormat=Timeseries  SampleTime=-1
      settings: Description=|
      | jointCommand
      | 
      | WHAT THIS BLOCK DOES
      | Records the input as a MATLAB timeseries for plots and validation. It does not feed a control action back to the robot.
      | 
      | FOLDER CONTEXT
      | RESULTS AND RECORDINGS
      | 
      | Purpose: record signals for plotting and comparison. These blocks do not control the robot.
      | trueState: actual motion; estimatedState: observer output; jointCommand: applied targets.
      | sensorReadout, worldPush and balanceCorrection complete the experiment records.
  sensorReadout : ToWorkspace  VariableName=sensorReadout  SaveFormat=Timeseries  SampleTime=-1
      settings: Description=|
      | sensorReadout
      | 
      | WHAT THIS BLOCK DOES
      | Records the input as a MATLAB timeseries for plots and validation. It does not feed a control action back to the robot.
      | 
      | FOLDER CONTEXT
      | RESULTS AND RECORDINGS
      | 
      | Purpose: record signals for plotting and comparison. These blocks do not control the robot.
      | trueState: actual motion; estimatedState: observer output; jointCommand: applied targets.
      | sensorReadout, worldPush and balanceCorrection complete the experiment records.
  trueState : ToWorkspace  VariableName=trueState  SaveFormat=Timeseries  SampleTime=-1
      settings: Description=|
      | trueState
      | 
      | WHAT THIS BLOCK DOES
      | Records the input as a MATLAB timeseries for plots and validation. It does not feed a control action back to the robot.
      | 
      | FOLDER CONTEXT
      | RESULTS AND RECORDINGS
      | 
      | Purpose: record signals for plotting and comparison. These blocks do not control the robot.
      | trueState: actual motion; estimatedState: observer output; jointCommand: applied targets.
      | sensorReadout, worldPush and balanceCorrection complete the experiment records.
  worldPush : ToWorkspace  VariableName=worldPush  SaveFormat=Timeseries  SampleTime=-1
      settings: Description=|
      | worldPush
      | 
      | WHAT THIS BLOCK DOES
      | Records the input as a MATLAB timeseries for plots and validation. It does not feed a control action back to the robot.
      | 
      | FOLDER CONTEXT
      | RESULTS AND RECORDINGS
      | 
      | Purpose: record signals for plotting and comparison. These blocks do not control the robot.
      | trueState: actual motion; estimatedState: observer output; jointCommand: applied targets.
      | sensorReadout, worldPush and balanceCorrection complete the experiment records.
  wires:
  [md8_balanceCorrection] -> balanceCorrection/1
  [md8_estimatedState] -> estimatedState/1
  [md8_jointCommand] -> jointCommand/1
  [md8_sensorReadout] -> sensorReadout/1
  [md8_trueState] -> trueState/1
  [md8_worldPush] -> worldPush/1

== system microduck_nonlinear_state_feedback/Robot plant ==
  note: ROBOT PLANT
      |
      | Purpose: predict how the robot moves when its eight servo targets change.
      | Read the folders for motor torque, body motion, ground forces and sensors.
      | Inputs are desired joint angles; outputs are true states, sensor readings and the test push.
  Joint targets u - rad : Inport  Description=|
      | Joint targets u - rad
      | 
      | WHAT THIS BLOCK DOES
      | Receives this named signal from the parent folder. Check the name for its meaning and units.
      | 
      | FOLDER CONTEXT
      | ROBOT PLANT
      | 
      | Purpose: predict how the robot moves when its eight servo targets change.
      | Read the folders for motor torque, body motion, ground forces and sensors.
      | Inputs are desired joint angles; outputs are true states, sensor readings and the test push.
  External torso push : Subsystem  Description=|
      | EXTERNAL TORSO PUSH
      | 
      | Purpose: supply the repeatable disturbance used in this experiment.
      | A Gaussian 0.1 N forward push peaks at 0.2 s, with width 0.02 s.
      | It acts at the torso origin; the observer is not told this disturbance.
      mask help:
      | EXTERNAL TORSO PUSH
      |
      | Purpose: supply the repeatable disturbance used in this experiment.
      | A Gaussian 0.1 N forward push peaks at 0.2 s, with width 0.02 s.
      | It acts at the torso origin; the observer is not told this disturbance.
      settings: OpenFcn=open_system(gcb,'force');
      mask Display: disp('External torso push');
  Full state q v tau : Mux  Description=|  Inputs=3
      | Full state q v tau
      | 
      | WHAT THIS BLOCK DOES
      | Joins the input vectors in port order, top to bottom. This packages signals; it does not add forces or mix units.
      | 
      | FOLDER CONTEXT
      | ROBOT PLANT
      | 
      | Purpose: predict how the robot moves when its eight servo targets change.
      | Read the folders for motor torque, body motion, ground forces and sensors.
      | Inputs are desired joint angles; outputs are true states, sensor readings and the test push.
  Ground contact : Subsystem  Description=|
      | GROUND CONTACT
      | 
      | Purpose: calculate how the floor pushes on the two feet.
      | There are four sole points per foot. Open one point to see its spring, damper and friction law.
      | Add their eight generalized force vectors to obtain the total ground contribution.
      mask help:
      | GROUND CONTACT
      |
      | Purpose: calculate how the floor pushes on the two feet.
      | There are four sole points per foot. Open one point to see its spring, damper and friction law.
      | Add their eight generalized force vectors to obtain the total ground contribution.
      settings: OpenFcn=open_system(gcb,'force');
      mask Display: disp('Ground contact');
  IMU and encoders : Subsystem  Description=|
      | IMU AND ENCODERS
      | 
      | Purpose: predict the readings available to the observer.
      | Gyro = R transpose * world angular velocity. Specific force subtracts gravity and includes IMU offset.
      | Rotate to trunk axes, then append eight joint angles. No true torso angles are measured directly.
      mask help:
      | IMU AND ENCODERS
      |
      | Purpose: predict the readings available to the observer.
      | Gyro = R transpose * world angular velocity. Specific force subtracts gravity and includes IMU offset.
      | Rotate to trunk axes, then append eight joint angles. No true torso angles are measured directly.
      settings: OpenFcn=open_system(gcb,'force');
      mask Display: disp('IMU and encoders');
  Integrate body motion : Subsystem  Description=|
      | INTEGRATE BODY MOTION
      | 
      | Purpose: convert generalized acceleration into the robot pose over time.
      | First integrator: acceleration -> velocity v. Second integrator: velocity -> coordinates q.
      | The initial pose is the trimmed standing equilibrium. q and v each contain 14 values.
      mask help:
      | INTEGRATE BODY MOTION
      |
      | Purpose: convert generalized acceleration into the robot pose over time.
      | First integrator: acceleration -> velocity v. Second integrator: velocity -> coordinates q.
      | The initial pose is the trimmed standing equilibrium. q and v each contain 14 values.
      settings: OpenFcn=open_system(gcb,'force');
      mask Display: disp('Integrate body motion');
  Rigid body force balance : Subsystem  Description=|
      | RIGID BODY FORCE BALANCE
      | 
      | Purpose: combine all physical forces and solve for acceleration.
      | M * acceleration = motor + contact + push - gravity and velocity bias - damping.
      | M couples the body and joints, so acceleration is found with one matrix solve.
      mask help:
      | RIGID BODY FORCE BALANCE
      |
      | Purpose: combine all physical forces and solve for acceleration.
      | M * acceleration = motor + contact + push - gravity and velocity bias - damping.
      | M couples the body and joints, so acceleration is found with one matrix solve.
      settings: OpenFcn=open_system(gcb,'force');
      mask Display: disp('Rigid body force balance');
  Servo position control : Subsystem  Description=|
      | SERVO POSITION CONTROL
      | 
      | Purpose: model the eight internal position servos, including their response delay.
      | Angle error -> internal PD torque -> torque limit -> first-order torque lag.
      | These inner loops are part of the plant; the outer balance PID changes their targets.
      mask help:
      | SERVO POSITION CONTROL
      |
      | Purpose: model the eight internal position servos, including their response delay.
      | Angle error -> internal PD torque -> torque limit -> first-order torque lag.
      | These inner loops are part of the plant; the outer balance PID changes their targets.
      settings: OpenFcn=open_system(gcb,'force');
      mask Display: disp('Servo position control');
  True state x - 36 : Outport  Description=|
      | True state x - 36
      | 
      | WHAT THIS BLOCK DOES
      | Carries this named result out of the folder. The port number defines the interface order.
      | 
      | FOLDER CONTEXT
      | ROBOT PLANT
      | 
      | Purpose: predict how the robot moves when its eight servo targets change.
      | Read the folders for motor torque, body motion, ground forces and sensors.
      | Inputs are desired joint angles; outputs are true states, sensor readings and the test push.
  Sensors y - 14 : Outport  Description=|  Port=2
      | Sensors y - 14
      | 
      | WHAT THIS BLOCK DOES
      | Carries this named result out of the folder. The port number defines the interface order.
      | 
      | FOLDER CONTEXT
      | ROBOT PLANT
      | 
      | Purpose: predict how the robot moves when its eight servo targets change.
      | Read the folders for motor torque, body motion, ground forces and sensors.
      | Inputs are desired joint angles; outputs are true states, sensor readings and the test push.
  Test wrench w - 6 : Outport  Description=|  Port=3
      | Test wrench w - 6
      | 
      | WHAT THIS BLOCK DOES
      | Carries this named result out of the folder. The port number defines the interface order.
      | 
      | FOLDER CONTEXT
      | ROBOT PLANT
      | 
      | Purpose: predict how the robot moves when its eight servo targets change.
      | Read the folders for motor torque, body motion, ground forces and sensors.
      | Inputs are desired joint angles; outputs are true states, sensor readings and the test push.
  wires:
  Integrate body motion/1(Out1) -> Full state q v tau/1, Servo position control/2(Coordinates q)
  Integrate body motion/3(Out3) -> Full state q v tau/2, Servo position control/3(Velocities v)
  Servo position control/1(Actual torques tau - Nm) -> Full state q v tau/3, Rigid body force balance/2(Motor torques)
  Integrate body motion/2(Out2) -> Ground contact/1(Pose and velocity), IMU and encoders/1(Pose and velocity), Rigid body force balance/1(Pose and velocity)
  Rigid body force balance/1(Acceleration - 14) -> IMU and encoders/2(Generalized acceleration), Integrate body motion/1(In1)
  Ground contact/1(Ground forces - 14) -> Rigid body force balance/3(Ground forces)
  External torso push/1(World wrench w - 6) -> Rigid body force balance/4(External wrench), Test wrench w - 6/1
  Joint targets u - rad/1 -> Servo position control/1(Desired angles u)
  Full state q v tau/1 -> True state x - 36/1
  IMU and encoders/1(Gyro accel encoders - 14) -> Sensors y - 14/1

== system microduck_nonlinear_state_feedback/State feedback controller ==
  note: LECTURE 9: STATE FEEDBACK BY POLE PLACEMENT
      | u = ueq - K S^{-1}(xhat-xeq)
      | Choose requested closed-loop poles, then calculate K using place.
      | The existing fast stable plant modes are retained; no LQR weighting matrices.
      | Standing regulation; no extra integral/reference-tracking states in this experiment.
  Retained state x or xhat - 33 : Inport
  Deviation from standing : Sum  Inputs=+-
  Hold joint targets between samples : ZeroOrderHold  Description=Digital controller period Ts. Its input is sampled at the same period as the observer and true-state baseline.  SampleTime=r.observer.sampleTime
  Joint command limits : Saturate  Description=Same eight absolute joint-command limits as the PID plant experiment. Applied command feeds the plant AND observer predictor.  UpperLimit=r.p.jointMax  LowerLimit=r.p.jointMin
  Limit state feedback corrections : Saturate  Description=Limit each of the eight joint-angle offsets. Compare requested/limited values to detect clipping. There is no integrator to wind up.  UpperLimit=r.feedback.maxCorrectionRad  LowerLimit=-r.feedback.maxCorrectionRad
  Normalize physical states : Gain  Description=z = S^(-1)*(x-xeq). Scaling makes metres, radians, rates and torques comparable in the LQR cost.  Gain=inv(r.observer.S)  Multiplication=Matrix(K*u)
  Pole placement negative state feedback : Gain  Description=du = -K*z. K is calculated using pole placement in equivalent state coordinates; no LQR cost or weights are used.  Gain=-r.feedback.K  Multiplication=Matrix(K*u)
  Standing joint targets : Constant  Value=r.p.ueq
  Standing retained state : Constant  Value=r.p.xeq(r.observer.keep)
  Standing targets plus correction : Sum
  Desired joint angles u - 8 : Outport
  Joint corrections du - 8 : Outport  Port=2
  wires:
  Retained state x or xhat - 33/1 -> Deviation from standing/1
  Standing retained state/1 -> Deviation from standing/2
  Deviation from standing/1 -> Normalize physical states/1
  Normalize physical states/1 -> Pole placement negative state feedback/1
  Pole placement negative state feedback/1 -> Limit state feedback corrections/1
  Limit state feedback corrections/1 -> Standing targets plus correction/1, Joint corrections du - 8/1
  Standing joint targets/1 -> Standing targets plus correction/2
  Standing targets plus correction/1 -> Joint command limits/1
  Joint command limits/1 -> Hold joint targets between samples/1
  Hold joint targets between samples/1 -> Desired joint angles u - 8/1

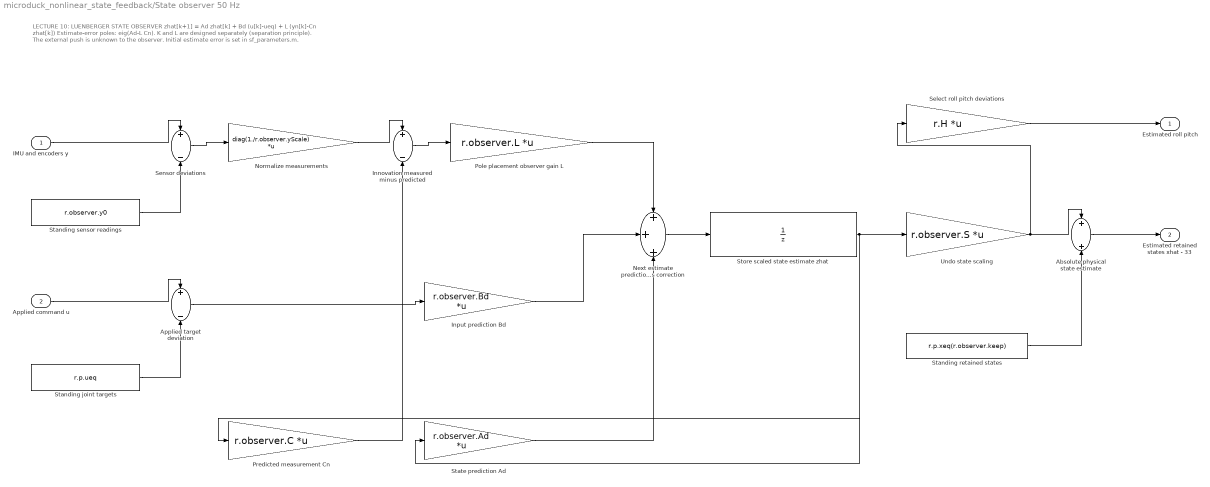
== system microduck_nonlinear_state_feedback/State observer 50 Hz ==
  note: LECTURE 10: LUENBERGER STATE OBSERVER
      | zhat[k+1] = Ad zhat[k] + Bd (u[k]-ueq) + L (yn[k]-Cn zhat[k])
      | Estimate-error poles: eig(Ad-L Cn). K and L are designed separately (separation principle).
      | The external push is unknown to the observer. Initial estimate error is set in sf_parameters.m.
  IMU and encoders y : Inport
  Applied command u : Inport  Port=2
  Absolute physical state estimate : Sum
  Applied target deviation : Sum  Inputs=+-
  Innovation measured minus predicted : Sum  Inputs=+-
  Input prediction Bd : Gain  Description=Bd*(u_applied-ueq). The known input includes outer-controller command limiting.  Gain=r.observer.Bd  Multiplication=Matrix(K*u)
  Next estimate prediction plus correction : Sum  Inputs=+++
  Normalize measurements : Gain  Description=yn = diag(1./yScale)*(y-yeq). Same physical sensors and normalization as the earlier plant.  Gain=diag(1./r.observer.yScale)  Multiplication=Matrix(K*u)
  Pole placement observer gain L : Gain  Description=L*innovation. L is designed by pole placement on the dual system, not by a Kalman filter or covariance weights.  Gain=r.observer.L  Multiplication=Matrix(K*u)
  Predicted measurement Cn : Gain  Gain=r.observer.C  Multiplication=Matrix(K*u)
  Select roll pitch deviations : Gain  Gain=r.H  Multiplication=Matrix(K*u)
  Sensor deviations : Sum  Inputs=+-
  Standing joint targets : Constant  Value=r.p.ueq
  Standing retained states : Constant  Value=r.p.xeq(r.observer.keep)
  Standing sensor readings : Constant  Value=r.observer.y0
  State prediction Ad : Gain  Gain=r.observer.Ad  Multiplication=Matrix(K*u)
  Store scaled state estimate zhat : UnitDelay  Description=Stores zhat[k]. Its input becomes zhat[k+1] at the next sample. This delay makes the observer causal.  InitialCondition=r.observer.S\r.observer.settings.initialEstimateDelta(r.observer.keep)  SampleTime=r.observer.sampleTime
  Undo state scaling : Gain  Gain=r.observer.S  Multiplication=Matrix(K*u)
  Estimated roll pitch : Outport
  Estimated retained states xhat - 33 : Outport  Port=2
  wires:
  IMU and encoders y/1 -> Sensor deviations/1
  Standing sensor readings/1 -> Sensor deviations/2
  Sensor deviations/1 -> Normalize measurements/1
  Normalize measurements/1 -> Innovation measured minus predicted/1
  Predicted measurement Cn/1 -> Innovation measured minus predicted/2
  Innovation measured minus predicted/1 -> Pole placement observer gain L/1
  Applied command u/1 -> Applied target deviation/1
  Standing joint targets/1 -> Applied target deviation/2
  Applied target deviation/1 -> Input prediction Bd/1
  Input prediction Bd/1 -> Next estimate prediction plus correction/2
  Pole placement observer gain L/1 -> Next estimate prediction plus correction/1
  State prediction Ad/1 -> Next estimate prediction plus correction/3
  Next estimate prediction plus correction/1 -> Store scaled state estimate zhat/1
  Store scaled state estimate zhat/1 -> State prediction Ad/1, Predicted measurement Cn/1, Undo state scaling/1
  Undo state scaling/1 -> Absolute physical state estimate/1, Select roll pitch deviations/1
  Standing retained states/1 -> Absolute physical state estimate/2
  Absolute physical state estimate/1 -> Estimated retained states xhat - 33/1
  Select roll pitch deviations/1 -> Estimated roll pitch/1

== system microduck_nonlinear_state_feedback/Robot plant/External torso push ==
  note: EXTERNAL TORSO PUSH
      |
      | Purpose: supply the repeatable disturbance used in this experiment.
      | A Gaussian 0.1 N forward push peaks at 0.2 s, with width 0.02 s.
      | It acts at the torso origin; the observer is not told this disturbance.
  Gaussian push envelope : Fcn  Description=|  Expr=exp(-((u-r.test.pushCentre)/r.test.pushWidth)^2)
      | Gaussian push envelope
      | 
      | WHAT THIS BLOCK DOES
      | Performs the mathematical operation named on this block. Open its parameter dialog to inspect the operator and dimensions.
      | 
      | FOLDER CONTEXT
      | EXTERNAL TORSO PUSH
      | 
      | Purpose: supply the repeatable disturbance used in this experiment.
      | A Gaussian 0.1 N forward push peaks at 0.2 s, with width 0.02 s.
      | It acts at the torso origin; the observer is not told this disturbance.
  Time : Clock
      settings: Description=|
      | Time
      | 
      | WHAT THIS BLOCK DOES
      | Performs the mathematical operation named on this block. Open its parameter dialog to inspect the operator and dimensions.
      | 
      | FOLDER CONTEXT
      | EXTERNAL TORSO PUSH
      | 
      | Purpose: supply the repeatable disturbance used in this experiment.
      | A Gaussian 0.1 N forward push peaks at 0.2 s, with width 0.02 s.
      | It acts at the torso origin; the observer is not told this disturbance.
  World force and moment amplitudes : Gain  Description=|  Gain=push_wrench  Multiplication=Matrix(K*u)
      | SHARED PARAMETER: push_wrench = [r.test.pushForce;r.test.pushMoment]
      | Edit sf_parameters.m; per-model edits are refreshed on Run.
      | 
      | WHAT THIS BLOCK DOES
      | World force and moment amplitudes
      | 
      | PARAMETER
      | G10 = [r.test.pushForce;zeros(3,1)]
      | 
      | The short symbol is stored in this model workspace. Its numeric value is unchanged from the validated model.
  World wrench w - 6 : Outport  Description=|
      | World wrench w - 6
      | 
      | WHAT THIS BLOCK DOES
      | Carries this named result out of the folder. The port number defines the interface order.
      | 
      | FOLDER CONTEXT
      | EXTERNAL TORSO PUSH
      | 
      | Purpose: supply the repeatable disturbance used in this experiment.
      | A Gaussian 0.1 N forward push peaks at 0.2 s, with width 0.02 s.
      | It acts at the torso origin; the observer is not told this disturbance.
  wires:
  Time/1 -> Gaussian push envelope/1
  Gaussian push envelope/1 -> World force and moment amplitudes/1
  World force and moment amplitudes/1 -> World wrench w - 6/1

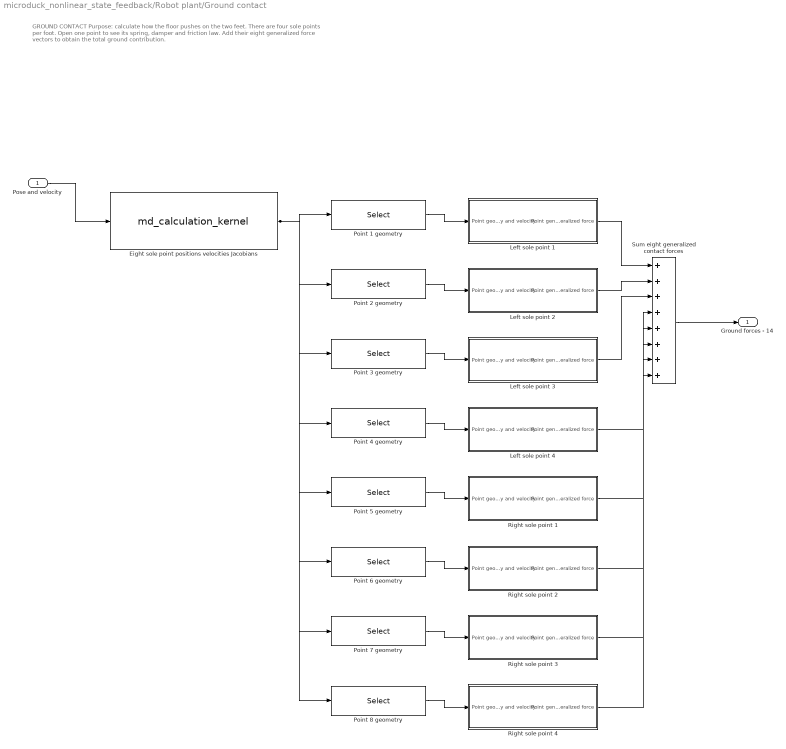
== system microduck_nonlinear_state_feedback/Robot plant/Ground contact ==
  note: GROUND CONTACT
      |
      | Purpose: calculate how the floor pushes on the two feet.
      | There are four sole points per foot. Open one point to see its spring, damper and friction law.
      | Add their eight generalized force vectors to obtain the total ground contribution.
  Pose and velocity : Inport  Description=|
      | Pose and velocity
      | 
      | WHAT THIS BLOCK DOES
      | Receives this named signal from the parent folder. Check the name for its meaning and units.
      | 
      | FOLDER CONTEXT
      | GROUND CONTACT
      | 
      | Purpose: calculate how the floor pushes on the two feet.
      | There are four sole points per foot. Open one point to see its spring, damper and friction law.
      | Add their eight generalized force vectors to obtain the total ground contribution.
  Eight sole point positions velocities Jacobians : M-S-Function  Description=|  FunctionName=md_calculation_kernel  Parameters=r.p, 'points'
      | Eight sole point positions velocities Jacobians
      | 
      | WHAT THIS BLOCK DOES
      | Performs the mathematical operation named on this block. Open its parameter dialog to inspect the operator and dimensions.
      | 
      | FOLDER CONTEXT
      | GROUND CONTACT
      | 
      | Purpose: calculate how the floor pushes on the two feet.
      | There are four sole points per foot. Open one point to see its spring, damper and friction law.
      | Add their eight generalized force vectors to obtain the total ground contribution.
      settings: OpenFcn=edit md_rigid_body_math; edit md_calculation_kernel;
  Left sole point 1 : Subsystem  Description=|
      | LEFT SOLE POINT 1
      | 
      | Purpose: calculate the floor force at one sole corner.
      | If z < 0: fn = max(0, -kn*z - cn*vz); otherwise fn = 0.
      | Friction opposes horizontal slip. J transpose maps the point force into 14 generalized forces.
      mask help:
      | LEFT SOLE POINT 1
      |
      | Purpose: calculate the floor force at one sole corner.
      | If z < 0: fn = max(0, -kn*z - cn*vz); otherwise fn = 0.
      | Friction opposes horizontal slip. J transpose maps the point force into 14 generalized forces.
      settings: OpenFcn=open_system(gcb,'force');
      mask Display: disp('Left sole point 1');
  Left sole point 2 : Subsystem  Description=|
      | LEFT SOLE POINT 2
      | 
      | Purpose: calculate the floor force at one sole corner.
      | If z < 0: fn = max(0, -kn*z - cn*vz); otherwise fn = 0.
      | Friction opposes horizontal slip. J transpose maps the point force into 14 generalized forces.
      mask help:
      | LEFT SOLE POINT 2
      |
      | Purpose: calculate the floor force at one sole corner.
      | If z < 0: fn = max(0, -kn*z - cn*vz); otherwise fn = 0.
      | Friction opposes horizontal slip. J transpose maps the point force into 14 generalized forces.
      settings: OpenFcn=open_system(gcb,'force');
      mask Display: disp('Left sole point 2');
  Left sole point 3 : Subsystem  Description=|
      | LEFT SOLE POINT 3
      | 
      | Purpose: calculate the floor force at one sole corner.
      | If z < 0: fn = max(0, -kn*z - cn*vz); otherwise fn = 0.
      | Friction opposes horizontal slip. J transpose maps the point force into 14 generalized forces.
      mask help:
      | LEFT SOLE POINT 3
      |
      | Purpose: calculate the floor force at one sole corner.
      | If z < 0: fn = max(0, -kn*z - cn*vz); otherwise fn = 0.
      | Friction opposes horizontal slip. J transpose maps the point force into 14 generalized forces.
      settings: OpenFcn=open_system(gcb,'force');
      mask Display: disp('Left sole point 3');
  Left sole point 4 : Subsystem  Description=|
      | LEFT SOLE POINT 4
      | 
      | Purpose: calculate the floor force at one sole corner.
      | If z < 0: fn = max(0, -kn*z - cn*vz); otherwise fn = 0.
      | Friction opposes horizontal slip. J transpose maps the point force into 14 generalized forces.
      mask help:
      | LEFT SOLE POINT 4
      |
      | Purpose: calculate the floor force at one sole corner.
      | If z < 0: fn = max(0, -kn*z - cn*vz); otherwise fn = 0.
      | Friction opposes horizontal slip. J transpose maps the point force into 14 generalized forces.
      settings: OpenFcn=open_system(gcb,'force');
      mask Display: disp('Left sole point 4');
  Point 1 geometry : Selector  Description=|  InputPortWidth=384  IndexOptions=Index vector (dialog)  Indices=[1 2 3 4 5 6 7 8 9 10 11 12 13 14 15 16 17 18 19 20 21 22 23 24 25 26 27 28 29 30 31 32 33 34 35 36 37 38 39 40 41 42 43 44 45 46 47 48]  OutputSizes=1
      | Point 1 geometry
      | 
      | WHAT THIS BLOCK DOES
      | Selects the labelled coordinates from an input vector without changing their physical values. Open the block to see the one-based index list.
      | 
      | FOLDER CONTEXT
      | GROUND CONTACT
      | 
      | Purpose: calculate how the floor pushes on the two feet.
      | There are four sole points per foot. Open one point to see its spring, damper and friction law.
      | Add their eight generalized force vectors to obtain the total ground contribution.
  Point 2 geometry : Selector  Description=|  InputPortWidth=384  IndexOptions=Index vector (dialog)  Indices=[49 50 51 52 53 54 55 56 57 58 59 60 61 62 63 64 65 66 67 68 69 70 71 72 73 74 75 76 77 78 79 80 81 82 83 84 85 86 87 88 89 90 91 92 93 94 95 96]  OutputSizes=1
      | Point 2 geometry
      | 
      | WHAT THIS BLOCK DOES
      | Selects the labelled coordinates from an input vector without changing their physical values. Open the block to see the one-based index list.
      | 
      | FOLDER CONTEXT
      | GROUND CONTACT
      | 
      | Purpose: calculate how the floor pushes on the two feet.
      | There are four sole points per foot. Open one point to see its spring, damper and friction law.
      | Add their eight generalized force vectors to obtain the total ground contribution.
  Point 3 geometry : Selector  Description=|  InputPortWidth=384  IndexOptions=Index vector (dialog)  Indices=[97 98 99 100 101 102 103 104 105 106 107 108 109 110 111 112 113 114 115 116 117 118 119 120 121 122 123 124 125 126 127 128 129 130 131 132 133 134 135 136 137 138 139 140 141 142 143 144]  OutputSizes=1
      | Point 3 geometry
      | 
      | WHAT THIS BLOCK DOES
      | Selects the labelled coordinates from an input vector without changing their physical values. Open the block to see the one-based index list.
      | 
      | FOLDER CONTEXT
      | GROUND CONTACT
      | 
      | Purpose: calculate how the floor pushes on the two feet.
      | There are four sole points per foot. Open one point to see its spring, damper and friction law.
      | Add their eight generalized force vectors to obtain the total ground contribution.
  Point 4 geometry : Selector  Description=|  InputPortWidth=384  IndexOptions=Index vector (dialog)  Indices=[145 146 147 148 149 150 151 152 153 154 155 156 157 158 159 160 161 162 163 164 165 166 167 168 169 170 171 172 173 174 175 176 177 178 179 180 181 182 183 184 185 186 187 188 189 190 191 192]  OutputSizes=1
      | Point 4 geometry
      | 
      | WHAT THIS BLOCK DOES
      | Selects the labelled coordinates from an input vector without changing their physical values. Open the block to see the one-based index list.
      | 
      | FOLDER CONTEXT
      | GROUND CONTACT
      | 
      | Purpose: calculate how the floor pushes on the two feet.
      | There are four sole points per foot. Open one point to see its spring, damper and friction law.
      | Add their eight generalized force vectors to obtain the total ground contribution.
  Point 5 geometry : Selector  Description=|  InputPortWidth=384  IndexOptions=Index vector (dialog)  Indices=[193 194 195 196 197 198 199 200 201 202 203 204 205 206 207 208 209 210 211 212 213 214 215 216 217 218 219 220 221 222 223 224 225 226 227 228 229 230 231 232 233 234 235 236 237 238 239 240]  OutputSizes=1
      | Point 5 geometry
      | 
      | WHAT THIS BLOCK DOES
      | Selects the labelled coordinates from an input vector without changing their physical values. Open the block to see the one-based index list.
      | 
      | FOLDER CONTEXT
      | GROUND CONTACT
      | 
      | Purpose: calculate how the floor pushes on the two feet.
      | There are four sole points per foot. Open one point to see its spring, damper and friction law.
      | Add their eight generalized force vectors to obtain the total ground contribution.
  Point 6 geometry : Selector  Description=|  InputPortWidth=384  IndexOptions=Index vector (dialog)  Indices=[241 242 243 244 245 246 247 248 249 250 251 252 253 254 255 256 257 258 259 260 261 262 263 264 265 266 267 268 269 270 271 272 273 274 275 276 277 278 279 280 281 282 283 284 285 286 287 288]  OutputSizes=1
      | Point 6 geometry
      | 
      | WHAT THIS BLOCK DOES
      | Selects the labelled coordinates from an input vector without changing their physical values. Open the block to see the one-based index list.
      | 
      | FOLDER CONTEXT
      | GROUND CONTACT
      | 
      | Purpose: calculate how the floor pushes on the two feet.
      | There are four sole points per foot. Open one point to see its spring, damper and friction law.
      | Add their eight generalized force vectors to obtain the total ground contribution.
  Point 7 geometry : Selector  Description=|  InputPortWidth=384  IndexOptions=Index vector (dialog)  Indices=[289 290 291 292 293 294 295 296 297 298 299 300 301 302 303 304 305 306 307 308 309 310 311 312 313 314 315 316 317 318 319 320 321 322 323 324 325 326 327 328 329 330 331 332 333 334 335 336]  OutputSizes=1
      | Point 7 geometry
      | 
      | WHAT THIS BLOCK DOES
      | Selects the labelled coordinates from an input vector without changing their physical values. Open the block to see the one-based index list.
      | 
      | FOLDER CONTEXT
      | GROUND CONTACT
      | 
      | Purpose: calculate how the floor pushes on the two feet.
      | There are four sole points per foot. Open one point to see its spring, damper and friction law.
      | Add their eight generalized force vectors to obtain the total ground contribution.
  Point 8 geometry : Selector  Description=|  InputPortWidth=384  IndexOptions=Index vector (dialog)  Indices=[337 338 339 340 341 342 343 344 345 346 347 348 349 350 351 352 353 354 355 356 357 358 359 360 361 362 363 364 365 366 367 368 369 370 371 372 373 374 375 376 377 378 379 380 381 382 383 384]  OutputSizes=1
      | Point 8 geometry
      | 
      | WHAT THIS BLOCK DOES
      | Selects the labelled coordinates from an input vector without changing their physical values. Open the block to see the one-based index list.
      | 
      | FOLDER CONTEXT
      | GROUND CONTACT
      | 
      | Purpose: calculate how the floor pushes on the two feet.
      | There are four sole points per foot. Open one point to see its spring, damper and friction law.
      | Add their eight generalized force vectors to obtain the total ground contribution.
  Right sole point 1 : Subsystem  Description=|
      | RIGHT SOLE POINT 1
      | 
      | Purpose: calculate the floor force at one sole corner.
      | If z < 0: fn = max(0, -kn*z - cn*vz); otherwise fn = 0.
      | Friction opposes horizontal slip. J transpose maps the point force into 14 generalized forces.
      mask help:
      | RIGHT SOLE POINT 1
      |
      | Purpose: calculate the floor force at one sole corner.
      | If z < 0: fn = max(0, -kn*z - cn*vz); otherwise fn = 0.
      | Friction opposes horizontal slip. J transpose maps the point force into 14 generalized forces.
      settings: OpenFcn=open_system(gcb,'force');
      mask Display: disp('Right sole point 1');
  Right sole point 2 : Subsystem  Description=|
      | RIGHT SOLE POINT 2
      | 
      | Purpose: calculate the floor force at one sole corner.
      | If z < 0: fn = max(0, -kn*z - cn*vz); otherwise fn = 0.
      | Friction opposes horizontal slip. J transpose maps the point force into 14 generalized forces.
      mask help:
      | RIGHT SOLE POINT 2
      |
      | Purpose: calculate the floor force at one sole corner.
      | If z < 0: fn = max(0, -kn*z - cn*vz); otherwise fn = 0.
      | Friction opposes horizontal slip. J transpose maps the point force into 14 generalized forces.
      settings: OpenFcn=open_system(gcb,'force');
      mask Display: disp('Right sole point 2');
  Right sole point 3 : Subsystem  Description=|
      | RIGHT SOLE POINT 3
      | 
      | Purpose: calculate the floor force at one sole corner.
      | If z < 0: fn = max(0, -kn*z - cn*vz); otherwise fn = 0.
      | Friction opposes horizontal slip. J transpose maps the point force into 14 generalized forces.
      mask help:
      | RIGHT SOLE POINT 3
      |
      | Purpose: calculate the floor force at one sole corner.
      | If z < 0: fn = max(0, -kn*z - cn*vz); otherwise fn = 0.
      | Friction opposes horizontal slip. J transpose maps the point force into 14 generalized forces.
      settings: OpenFcn=open_system(gcb,'force');
      mask Display: disp('Right sole point 3');
  Right sole point 4 : Subsystem  Description=|
      | RIGHT SOLE POINT 4
      | 
      | Purpose: calculate the floor force at one sole corner.
      | If z < 0: fn = max(0, -kn*z - cn*vz); otherwise fn = 0.
      | Friction opposes horizontal slip. J transpose maps the point force into 14 generalized forces.
      mask help:
      | RIGHT SOLE POINT 4
      |
      | Purpose: calculate the floor force at one sole corner.
      | If z < 0: fn = max(0, -kn*z - cn*vz); otherwise fn = 0.
      | Friction opposes horizontal slip. J transpose maps the point force into 14 generalized forces.
      settings: OpenFcn=open_system(gcb,'force');
      mask Display: disp('Right sole point 4');
  Sum eight generalized contact forces : Sum  Description=|  Inputs=++++++++
      | Sum eight generalized contact forces
      | 
      | WHAT THIS BLOCK DOES
      | Combines its inputs using the plus/minus signs shown on the icon. Signs: ++++++++.
      | 
      | FOLDER CONTEXT
      | GROUND CONTACT
      | 
      | Purpose: calculate how the floor pushes on the two feet.
      | There are four sole points per foot. Open one point to see its spring, damper and friction law.
      | Add their eight generalized force vectors to obtain the total ground contribution.
  Ground forces - 14 : Outport  Description=|
      | Ground forces - 14
      | 
      | WHAT THIS BLOCK DOES
      | Carries this named result out of the folder. The port number defines the interface order.
      | 
      | FOLDER CONTEXT
      | GROUND CONTACT
      | 
      | Purpose: calculate how the floor pushes on the two feet.
      | There are four sole points per foot. Open one point to see its spring, damper and friction law.
      | Add their eight generalized force vectors to obtain the total ground contribution.
  wires:
  Pose and velocity/1 -> Eight sole point positions velocities Jacobians/1
  Point 1 geometry/1 -> Left sole point 1/1(Point geometry and velocity)
  Point 2 geometry/1 -> Left sole point 2/1(Point geometry and velocity)
  Point 3 geometry/1 -> Left sole point 3/1(Point geometry and velocity)
  Point 4 geometry/1 -> Left sole point 4/1(Point geometry and velocity)
  Eight sole point positions velocities Jacobians/1 -> Point 1 geometry/1, Point 2 geometry/1, Point 3 geometry/1, Point 4 geometry/1, Point 5 geometry/1, Point 6 geometry/1, Point 7 geometry/1, Point 8 geometry/1
  Point 5 geometry/1 -> Right sole point 1/1(Point geometry and velocity)
  Point 6 geometry/1 -> Right sole point 2/1(Point geometry and velocity)
  Point 7 geometry/1 -> Right sole point 3/1(Point geometry and velocity)
  Point 8 geometry/1 -> Right sole point 4/1(Point geometry and velocity)
  Left sole point 1/1(Point generalized force) -> Sum eight generalized contact forces/1
  Left sole point 2/1(Point generalized force) -> Sum eight generalized contact forces/2
  Left sole point 3/1(Point generalized force) -> Sum eight generalized contact forces/3
  Left sole point 4/1(Point generalized force) -> Sum eight generalized contact forces/4
  Right sole point 1/1(Point generalized force) -> Sum eight generalized contact forces/5
  Right sole point 2/1(Point generalized force) -> Sum eight generalized contact forces/6
  Right sole point 3/1(Point generalized force) -> Sum eight generalized contact forces/7
  Right sole point 4/1(Point generalized force) -> Sum eight generalized contact forces/8
  Sum eight generalized contact forces/1 -> Ground forces - 14/1
